simulink model "tb_gnc_mission"  (R2026b)
settings: Solver=ode3  StopTime=10  FixedStep=1e-3  EnableMultiTasking=on
values from neighbouring files (symbols this model uses):
  cmd = y.get('gnc_cmd').Values    [gnc_mission_run.m]    (also in gnc_tb_run.m; t_gnc_mission.m = [1 2; 14 4; 26 5; 27 2; 32 7; 35 7])
  map = P.ic.Bus_TebMapInfo    [t_gnc_mission.m]    (also in t_t07_gnc_sil.m = struct())
  P = F.P    [gnc_fsm_driver.m]    (also in t_gnc_mission.m = r.P; t_t07_gnc_sil.m = shaddad_params('World', 3, 'Assign', false))
  Ts = pr.Ts    [t_gnc_mission.m]
undefined symbols (not defined in the file or in its folder): aligned, angles_B, bms_critical, charging, cmd_seq, DiscIntNeverNeededParam, drive_ready, estop_active, eul, gnssFixType, headingValid, heartbeat, implement_ready, implement_type, magnitude, navValid, pos_W, posStd, power_ready, protectiveStop, protFieldLen, quality, ranges_B, rc_link_ok, rc_mode_sw, scanValid, section_mask, SOC, t_scan, target_density, v_applied, v_track_meas, valid, vel_B, yawRate
libraries: simulink x15, robotmobilelib x1
settings Model: Creator=aomar  LastModifiedBy=aomar
settings ConfigSet: Description=Shaddad fixed-step 1 ms ode3, multitasking, explicit rate transitions (arch 7, D58).
settings OptimizationCC: SimCompilerOptimization=on
settings DebuggingCC: AlgebraicLoopMsg=error  ArtificialAlgebraicLoopMsg=error  SingleTaskRateTransMsg=error  StrictBusMsg=ErrorOnBusTreatedAsVector
settings SimscapeCC: SimscapeNominalValues="[{\"value\":\"1\",\"unit\":\"A\"},{\"value\":\"1\",\"unit\":\"bar\"},{\"value\":\"1\",\"unit\":\"cm^2\"},{\"value\":\"1\",\"unit\":\"cm^3/s\"},{\"value\":\"1\",\"unit\":\"kJ/kg\"},{\"value\":\"1\",\"unit\":\"kW\"},{\"value\":\"1\",\"unit\":\"l\"},{\"value\":\"1\",\"unit\":\"N\"},{\"value\":\"1\",\"unit\":\"N*m\"},{\"value\":\"1\",\"unit\":\"V\"},{\"value\":\"0.001\",\"unit\":\"Wb\"}]"  SimscapeNormalizeSystem=off  SimscapeUseEnergyAccounting=off

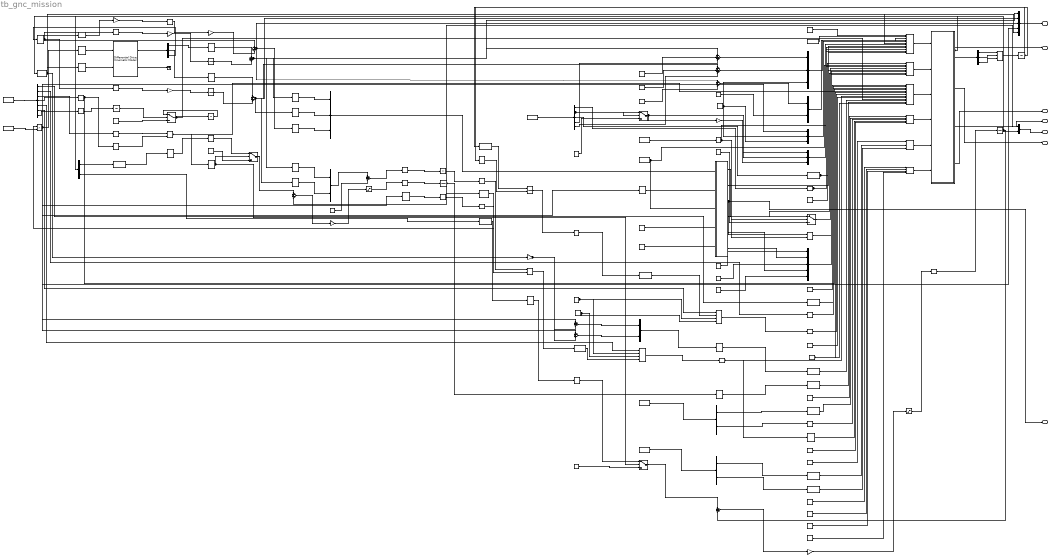
== system tb_gnc_mission ==
  BmsIC : Constant  Value=P.ic.Bus_BmsStatus  OutDataTypeStr=Bus: Bus_BmsStatus  SampleTime=Ts.hk
  BmsStatus : BusAssignment  AssignedSignals=SOC,bms_critical,charging,valid
  CmdIC : Constant  Value=P.ic.Bus_MissionCmd  OutDataTypeStr=Bus: Bus_MissionCmd  SampleTime=Ts.mcmd
  CmdSel : BusSelector  OutputSignals=v_cmd,omega_cmd
  GNC : ModelReference  ModelNameDialog=Shaddad_GNC  SimulationMode=Normal  ModelReferenceVersion=1.1
  HarnessLidar : MATLAB Function  TreatAsAtomicUnit=on  mask{prm=struct('res',P.world.occ.res,'origin',P.world.occ.origin,'rmin',P.sensors.lidar.rMin,'rmax',P.gnc.tb.lidar_rmax,'nBeams',P.gnc.obs.n_beams,'on',P.gnc.tb.lidar_on,'protXF',P.sensors.per.protXF,'protXR',P.sensors.per.protXR,'protL0',P.sensors.per.protL0,'protKv',P.sensors.per.protKv,'protW',P.sensors.per.protW,'protStatic',P.gnc.tb.prot_static,'mapN',P.gnc.map.local_N,'mapRes',P.gnc.map.local_res)}
  ImplSel : BusSelector  OutputSignals=mower_enable,tiller_enable,spray_enable
  Kinematics : robotmobilelib/Differential Drive Kinematic Model  VehicleInputs=Vehicle Speed & Heading Angular Velocity  WheelRadius=P.structure.r_sprocket  WheelSpeedRange=[-inf inf]  TrackWidth=P.structure.geom.B  InitialState=P.gnc.tb.x0(:)  SimulateUsing=Code generation
  Kv : Gain  Gain=P.electronics.shaper.K_v
  Kw : Gain  Gain=P.electronics.shaper.K_w_auto
  Map : BusCreator  Inputs=5  OutDataTypeStr=Bus: Bus_TebMapInfo  NonVirtualBus=on
  McuIC : Constant  Value=P.ic.Bus_McuStatus  OutDataTypeStr=Bus: Bus_McuStatus  SampleTime=Ts.gnc
  McuStatus : BusAssignment  AssignedSignals=rc_mode_sw,rc_link_ok,estop_active,drive_ready,power_ready,implement_ready,charging,implement_type,heartbeat,v_track_meas,v_applied,valid
  MissionCmd : BusAssignment  AssignedSignals=cmd,cmd_seq
  NavIC : Constant  Value=P.ic.Bus_NavState  OutDataTypeStr=Bus: Bus_NavState  SampleTime=Ts.ctrl
  NavState : BusAssignment  AssignedSignals=t,pos_W,eul,vel_B,yawRate,posStd,quality,navValid,headingValid,aligned,gnssFixType
  PerIC : Constant  Value=P.ic.Bus_Perception  OutDataTypeStr=Bus: Bus_Perception  SampleTime=Ts.lidar
  Perception : BusAssignment  AssignedSignals=t_scan,scanValid,ranges_B,angles_B,protectiveStop,protFieldLen,map
  RT_chg : RateTransition  OutPortSampleTime=Ts.hk
  RT_drive : RateTransition  OutPortSampleTime=Ts.ctrl
  RT_ppsi : RateTransition  OutPortSampleTime=Ts.lidar
  RT_pv : RateTransition  OutPortSampleTime=Ts.lidar
  RT_px : RateTransition  OutPortSampleTime=Ts.lidar
  RT_py : RateTransition  OutPortSampleTime=Ts.lidar
  RT_rc : RateTransition  OutPortSampleTime=0
  RT_v : RateTransition  OutPortSampleTime=Ts.ctrl
  RT_vLR : RateTransition  OutPortSampleTime=Ts.gnc
  RT_vapp : RateTransition  OutPortSampleTime=Ts.gnc
  RT_vc : RateTransition  OutPortSampleTime=0
  RT_vd : RateTransition  OutPortSampleTime=Ts.gnc
  RT_w : RateTransition  OutPortSampleTime=Ts.ctrl
  RT_xd : RateTransition  OutPortSampleTime=Ts.gnc
  RT_yd : RateTransition  OutPortSampleTime=Ts.gnc
  Spray : BusAssignment  AssignedSignals=section_mask,target_density,valid
  SprayIC : Constant  Value=P.ic.Bus_SprayDemand  OutDataTypeStr=Bus: Bus_SprayDemand  SampleTime=Ts.spray
  T_stateDot : Terminator
  ZOH_psi : RateTransition  OutPortSampleTime=Ts.ctrl
  ZOH_x : RateTransition  OutPortSampleTime=Ts.ctrl
  ZOH_y : RateTransition  OutPortSampleTime=Ts.ctrl
  a_sat : Saturate  UpperLimit=P.electronics.shaper.a_acc_auto  LowerLimit=-P.electronics.shaper.a_dec_auto
  al_sat : Saturate  UpperLimit=P.electronics.shaper.alpha_auto  LowerLimit=-P.electronics.shaper.alpha_auto
  at_dock : Logic  AllPortsSameDT=off  OutDataTypeStr=boolean
  at_dock_d : DataTypeConversion  OutDataTypeStr=double  RndMeth=Nearest
  bms_crit : simulink/Logic and Bit Operations/Compare To Constant  relop=>  const=0.5  OutDataTypeStr=boolean
  bms_d : Demux  Outputs=2
  bms_true : Constant  Value=true  OutDataTypeStr=boolean  SampleTime=Ts.hk
  charging : simulink/Logic and Bit Operations/Compare To Constant  relop=>  const=0.5  OutDataTypeStr=boolean
  chg_m : MultiPortSwitch  DataPortOrder=Zero-based contiguous  DiagnosticForDefault=None  zeroidx=on  SaturateOnIntegerOverflow=off  InputSameDT=off
  clock : DigitalClock  SampleTime=Ts.ctrl
  clock_l : DigitalClock  SampleTime=Ts.lidar
  cmd_d : Demux  Outputs=2
  cmd_u8 : DataTypeConversion  OutDataTypeStr=uint8  RndMeth=Nearest
  cmd_v : DataTypeConversion  OutDataTypeStr=double  RndMeth=Nearest
  cmd_w : DataTypeConversion  OutDataTypeStr=double  RndMeth=Nearest
  cos_psi : Trigonometry  Operator=cos
  ddock : Sum  Inputs=+-
  ddock2 : Math  Operator=magnitude^2
  ddock_s : Sum  Inputs=+
  dead_v : Delay  DelayLength=P.gnc.tb.n_dead  InitialCondition=0  SampleTime=Ts.ctrl
  dead_w : Delay  DelayLength=P.gnc.tb.n_dead  InitialCondition=0  SampleTime=Ts.ctrl
  dock_xy : Constant  Value=P.gnc.mission.dock(1:2)  OutDataTypeStr=double  SampleTime=Ts.gnc
  drift_x : Gain  Gain=-P.gnc.tb.drift
  drift_y : Gain  Gain=P.gnc.tb.drift
  drive_ok : Logic  AllPortsSameDT=off  OutDataTypeStr=boolean
  drv_rdy : simulink/Logic and Bit Operations/Compare To Constant  relop=>  const=0.5  OutDataTypeStr=boolean
  dx : DiscreteIntegrator  SampleTime=Ts.ctrl  ICPrevOutput=DiscIntNeverNeededParam  ICPrevScaledInput=DiscIntNeverNeededParam
  dy : DiscreteIntegrator  SampleTime=Ts.ctrl  ICPrevOutput=DiscIntNeverNeededParam  ICPrevScaledInput=DiscIntNeverNeededParam
  dyn : Constant  Value=P.gnc.tb.dyn  OutDataTypeStr=double
  estop : simulink/Logic and Bit Operations/Compare To Constant  relop=>  const=0.5  OutDataTypeStr=boolean
  eul : Mux  Inputs=[1 2]
  ev : Sum  Inputs=+-
  ew : Sum  Inputs=+-
  f0 : Constant  Value=0  OutDataTypeStr=double  SampleTime=Ts.gnc
  f1 : Constant  OutDataTypeStr=double  SampleTime=Ts.gnc
  freeze : simulink/Logic and Bit Operations/Compare To Constant  relop=>  const=0.5  OutDataTypeStr=boolean
  freeze_z : UnitDelay  InitialCondition=false  SampleTime=Ts.gnc
  gate_v : Switch  Criteria=u2 ~= 0  SaturateOnIntegerOverflow=off  InputSameDT=off
  gate_w : Switch  Criteria=u2 ~= 0  SaturateOnIntegerOverflow=off  InputSameDT=off
  hb : Switch  Criteria=u2 ~= 0  SaturateOnIntegerOverflow=off  InputSameDT=off
  hb_cnt : simulink/Sources/Counter Free-Running  NumBits=8  tsamp=Ts.gnc
  hb_z : UnitDelay  InitialCondition=uint8(0)  SampleTime=Ts.gnc
  impl_en : Logic  Operator=OR  Inputs=3  AllPortsSameDT=off  OutDataTypeStr=boolean
  impl_en_d : DataTypeConversion  OutDataTypeStr=double  RndMeth=Nearest
  impl_en_z : UnitDelay  InitialCondition=false  SampleTime=Ts.gnc
  impl_off : Logic  Operator=NOT  Inputs=1  AllPortsSameDT=off  OutDataTypeStr=boolean
  impl_rdy : simulink/Logic and Bit Operations/Compare To Constant  relop=>  const=0.5  OutDataTypeStr=boolean
  impl_rdy_m : MultiPortSwitch  DataPortOrder=Zero-based contiguous  DiagnosticForDefault=None  zeroidx=on  SaturateOnIntegerOverflow=off  InputSameDT=off
  impl_type : Constant  Value=P.gnc.mission.implement_type  OutDataTypeStr=uint8  SampleTime=Ts.gnc
  jerk_v : RateLimiter  RisingSlewLimit=P.electronics.shaper.j_max  FallingSlewLimit=-P.electronics.shaper.j_max  SampleTimeMode=inherited
  jerk_w : RateLimiter  RisingSlewLimit=P.electronics.shaper.jw_auto  FallingSlewLimit=-P.electronics.shaper.jw_auto  SampleTimeMode=inherited
  lag_r : simulink/Discrete/Transfer Fcn First Order  PoleZ=exp(-Ts.ctrl/P.gnc.tb.tau_r)  ICPrevOutput=0.0  DoSatur=off
  lag_v : simulink/Discrete/Transfer Fcn First Order  PoleZ=exp(-Ts.ctrl/P.gnc.tb.tau_v)  ICPrevOutput=0.0  DoSatur=off
  map_org : Constant  Value=-[1 1]*P.gnc.map.local_N/(2*P.gnc.map.local_res)  VectorParams1D=off  OutDataTypeStr=double  SampleTime=Ts.lidar
  map_res : Constant  Value=P.gnc.map.local_res  OutDataTypeStr=double  SampleTime=Ts.lidar
  map_size : Constant  Value=[1 1]*P.gnc.map.local_N  VectorParams1D=off  OutDataTypeStr=double  SampleTime=Ts.lidar
  mcu_d : Demux  Outputs=7
  mcu_true : Constant  Value=true  OutDataTypeStr=boolean  SampleTime=Ts.gnc
  n_psi : RandomNumber  Variance=P.gnc.tb.sig_yaw^2  Seed=P.gnc.tb.seed_psi  SampleTime=Ts.ctrl
  n_x : RandomNumber  Variance=P.gnc.tb.sig_pos^2  Seed=P.gnc.tb.seed_x  SampleTime=Ts.ctrl
  n_y : RandomNumber  Variance=P.gnc.tb.sig_pos^2  Seed=P.gnc.tb.seed_y  SampleTime=Ts.ctrl
  nan_r : Constant  Value=NaN(P.gnc.obs.n_beams, 1)  OutDataTypeStr=single  SampleTime=Ts.lidar
  nav_d : Demux  Outputs=5
  near_dock : simulink/Logic and Bit Operations/Compare To Constant  relop=<  const=P.gnc.tb.dock_tol^2  OutDataTypeStr=boolean
  no_estop : Logic  Operator=NOT  Inputs=1  AllPortsSameDT=off  OutDataTypeStr=boolean
  occ : Constant  Value=P.world.occ.grid  OutDataTypeStr=boolean
  posStd : Mux  Inputs=3
  pos_W : Mux  Inputs=3
  pose_l : Mux  Inputs=3
  prot_v : Logic  AllPortsSameDT=off  OutDataTypeStr=boolean
  psi_2pi : Gain  Gain=2*pi
  psi_b : Bias  Bias=pi  SaturateOnIntegerOverflow=off
  psi_f : Rounding
  psi_meas : Sum
  psi_n : Gain  Gain=1/(2*pi)
  psi_w : Sum  Inputs=+-
  quality : DataTypeConversion  OutDataTypeStr=uint8  RndMeth=Nearest
  ranges_v : Switch  Criteria=u2 ~= 0  SaturateOnIntegerOverflow=off  InputSameDT=off
  rc_link : simulink/Logic and Bit Operations/Compare To Constant  relop=>  const=0.5  OutDataTypeStr=boolean
  rc_sw : DataTypeConversion  OutDataTypeStr=uint8  RndMeth=Nearest
  scan_ok : simulink/Logic and Bit Operations/Compare To Constant  relop=>  const=0.5  OutDataTypeStr=boolean
  scn_bms : FromWorkspace  VariableName=P.gnc.tb.scn_bms  SampleTime=Ts.hk  OutputAfterFinalValue=Holding final value
  scn_cmd : FromWorkspace  VariableName=P.gnc.tb.scn_cmd  SampleTime=Ts.mcmd  Interpolate=off  OutputAfterFinalValue=Holding final value
  scn_mcu : FromWorkspace  VariableName=P.gnc.tb.scn_mcu  SampleTime=Ts.gnc  Interpolate=off  OutputAfterFinalValue=Holding final value
  scn_nav : FromWorkspace  VariableName=P.gnc.tb.scn_nav  SampleTime=Ts.ctrl  Interpolate=off  OutputAfterFinalValue=Holding final value
  scn_plant : FromWorkspace  VariableName=P.gnc.tb.scn_plant  SampleTime=Ts.ctrl  Interpolate=off  OutputAfterFinalValue=Holding final value
  scn_scan : FromWorkspace  VariableName=P.gnc.tb.scn_scan  SampleTime=Ts.lidar  Interpolate=off  OutputAfterFinalValue=Holding final value
  seq_u8 : DataTypeConversion  OutDataTypeStr=uint8  RndMeth=Nearest
  shaped_mux : Mux  Inputs=2
  sig : Switch  Criteria=u2 > Threshold  SaturateOnIntegerOverflow=off  InputSameDT=off
  sig_nom : Constant  Value=P.gnc.tb.sig_pos  OutDataTypeStr=double  SampleTime=Ts.ctrl
  sig_z : Gain  Gain=2
  sin_psi : Trigonometry
  soc_s : DataTypeConversion  OutDataTypeStr=single  RndMeth=Nearest
  spin_t : DiscreteIntegrator  ExternalReset=level  SampleTime=Ts.gnc  ICPrevOutput=DiscIntNeverNeededParam  ICPrevScaledInput=DiscIntNeverNeededParam
  spr_dens : Constant  Value=single(P.gnc.tb.spray_density)  OutDataTypeStr=single  SampleTime=Ts.spray
  spr_mask : Constant  Value=uint16(P.gnc.tb.spray_mask)  OutDataTypeStr=uint16  SampleTime=Ts.spray
  spr_valid : Constant  Value=true  OutDataTypeStr=boolean  SampleTime=Ts.spray
  spun : simulink/Logic and Bit Operations/Compare To Constant  relop=>=  const=P.gnc.tb.t_spin  OutDataTypeStr=boolean
  spun_d : DataTypeConversion  OutDataTypeStr=double  RndMeth=Nearest
  state : Demux  Outputs=3
  stopped : simulink/Logic and Bit Operations/Compare To Constant  relop=<  const=0.05  OutDataTypeStr=boolean
  tilt : Constant  Value=P.gnc.tb.tilt(:)  OutDataTypeStr=double  SampleTime=Ts.ctrl
  truth_mux : Mux  Inputs=5
  vL : Sum  Inputs=+-
  vLR : Mux  Inputs=2
  vLR_s : DataTypeConversion  OutDataTypeStr=single  RndMeth=Nearest
  vR : Sum
  v_abs : Abs  SaturateOnIntegerOverflow=off
  v_ref : DiscreteIntegrator  SampleTime=Ts.ctrl  ICPrevOutput=DiscIntNeverNeededParam  ICPrevScaledInput=DiscIntNeverNeededParam
  v_true : Product  Inputs=**
  valid : simulink/Logic and Bit Operations/Compare To Constant  relop=>  const=0.5  OutDataTypeStr=boolean
  vapp_s : DataTypeConversion  OutDataTypeStr=single  RndMeth=Nearest
  vel_B : Mux  Inputs=3
  w_ref : DiscreteIntegrator  SampleTime=Ts.ctrl  ICPrevOutput=DiscIntNeverNeededParam  ICPrevScaledInput=DiscIntNeverNeededParam
  w_track : Gain  Gain=P.electronics.mix.chi*P.electronics.mix.B/2
  x_meas : Sum  Inputs=+++
  x_true : Sum
  xy_t : Mux  Inputs=2
  y_meas : Sum  Inputs=+++
  y_true : Sum
  z_v : Constant  Value=0  OutDataTypeStr=double  SampleTime=Ts.ctrl
  z_w : Constant  Value=0  OutDataTypeStr=double  SampleTime=Ts.ctrl
  zero : Constant  Value=0  OutDataTypeStr=double  SampleTime=Ts.ctrl
  truth : Outport
  gnc_cmd : Outport  Port=2
  gnc_debug : Outport  Port=3
  gnc_status : Outport  Port=4
  shaped : Outport  Port=5
  nav_cmd : Outport  Port=6
  prot : Outport  Port=7
  wires:
  scn_mcu/1 -> mcu_d/1  "scn_mcu"
  scn_plant/1 -> v_true/2  "scn_plant"
  mcu_d/1 -> rc_sw/1  "scn_rc_sw"
  mcu_d/2 -> rc_link/1  "scn_rc_link"
  mcu_d/3 -> drv_rdy/1  "scn_drive_ready"
  mcu_d/4 -> estop/1  "scn_estop"
  mcu_d/5 -> chg_m/1  "scn_charging"
  mcu_d/6 -> impl_rdy_m/1  "scn_impl_ready"
  mcu_d/7 -> freeze/1  "scn_freeze"
  v_true/1 -> vR/1, vL/1, truth_mux/4, RT_vc/1, RT_vd/1, RT_pv/1, vel_B/1  "v_true"
  ZOH_psi/1 -> cos_psi/1, sin_psi/1, psi_w/1, psi_b/1  "ZOH_psi"
  lag_r/1 -> w_track/1, truth_mux/5, NavState/6, RT_rc/1  "r_true"
  CmdSel/1 -> cmd_v/1  "<v_cmd>"
  CmdSel/2 -> cmd_w/1  "<omega_cmd>"
  estop/1 -> no_estop/1, McuStatus/4  "estop"
  freeze/1 -> freeze_z/1  "freeze"
  psi_b/1 -> psi_n/1  "psi_b"
  RT_vc/1 -> Kinematics/1  "RT_vc"
  RT_rc/1 -> Kinematics/2  "RT_rc"
  psi_n/1 -> psi_f/1  "psi_n"
  sin_psi/1 -> drift_x/1  "sin_psi"
  cos_psi/1 -> drift_y/1  "cos_psi"
  hb_cnt/1 -> hb/3  "hb_cnt"
  drv_rdy/1 -> drive_ok/1  "drv_rdy"
  no_estop/1 -> drive_ok/2  "no_estop"
  freeze_z/1 -> hb/2  "freeze_z"
  cmd_v/1 -> RT_v/1  "cmd_v"
  Kinematics/1 -> state/1  "state"
  Kinematics/2 -> T_stateDot/1  "state_dot"
  state/1 -> ZOH_x/1  "state_1"
  state/2 -> ZOH_y/1  "state_2"
  state/3 -> ZOH_psi/1  "state_3"
  psi_f/1 -> psi_2pi/1  "psi_f"
  drift_x/1 -> dx/1  "drift_x"
  drift_y/1 -> dy/1  "drift_y"
  drive_ok/1 -> McuStatus/5, RT_drive/1  "drive_ok"
  RT_v/1 -> dead_v/1  "RT_v"
  hb/1 -> McuStatus/10, hb_z/1  "hb"
  psi_2pi/1 -> psi_w/2  "psi_2pi"
  z_v/1 -> gate_v/3  "z_v"
  dx/1 -> x_true/2  "dx"
  dy/1 -> y_true/2  "dy"
  hb_z/1 -> hb/1  "hb_z"
  dead_v/1 -> gate_v/1  "dead_v"
  ZOH_x/1 -> x_true/1  "ZOH_x"
  ZOH_y/1 -> y_true/1  "ZOH_y"
  RT_drive/1 -> gate_w/2, gate_v/2  "RT_drive"
  x_true/1 -> RT_xd/1, truth_mux/1, RT_px/1, x_meas/1  "x"
  y_true/1 -> RT_yd/1, truth_mux/2, y_meas/1, RT_py/1  "y"
  psi_w/1 -> RT_ppsi/1, psi_meas/1, truth_mux/3  "psi_w"
  gate_v/1 -> ev/1  "gate_v"
  ev/1 -> Kv/1  "ev"
  RT_px/1 -> pose_l/1  "RT_px"
  RT_py/1 -> pose_l/2  "RT_py"
  RT_ppsi/1 -> pose_l/3  "RT_ppsi"
  RT_xd/1 -> xy_t/1  "RT_xd"
  RT_yd/1 -> xy_t/2  "RT_yd"
  pose_l/1 -> HarnessLidar/1(pose)  "pose_l"
  xy_t/1 -> ddock/1  "xy_t"
  dock_xy/1 -> ddock/2  "dock_xy"
  Kv/1 -> a_sat/1  "Kv"
  ddock/1 -> ddock2/1  "ddock"
  a_sat/1 -> jerk_v/1  "a_sat"
  ddock2/1 -> ddock_s/1  "ddock2"
  jerk_v/1 -> v_ref/1  "jerk_v"
  RT_vd/1 -> v_abs/1  "RT_vd"
  ddock_s/1 -> near_dock/1  "ddock_s"
  v_abs/1 -> stopped/1  "v_abs"
  v_ref/1 -> RT_vapp/1, shaped_mux/1, ev/2, lag_v/1  "v_ref"
  impl_off/1 -> spin_t/2  "impl_off"
  near_dock/1 -> at_dock/1  "near_dock"
  stopped/1 -> at_dock/2  "stopped"
  lag_v/1 -> v_true/1  "lag_v"
  impl_en_d/1 -> spin_t/1  "impl_en_d"
  cmd_w/1 -> RT_w/1  "cmd_w"
  w_track/1 -> vR/2, vL/2  "w_track"
  at_dock/1 -> at_dock_d/1  "at_dock"
  spin_t/1 -> spun/1  "spin_t"
  RT_w/1 -> dead_w/1  "RT_w"
  scn_nav/1 -> nav_d/1  "scn_nav"
  nav_d/1 -> valid/1  "scn_valid"
  nav_d/2 -> sig/2, sig/1  "scn_sigma"
  nav_d/3 -> quality/1  "scn_quality"
  nav_d/4 -> x_meas/3  "scn_dx"
  nav_d/5 -> y_meas/3  "scn_dy"
  vL/1 -> vLR/1  "vL"
  vR/1 -> vLR/2  "vR"
  sig_nom/1 -> sig/3  "sig_nom"
  spun/1 -> spun_d/1  "spun"
  f0/1 -> chg_m/2, impl_rdy_m/3  "f0"
  z_w/1 -> gate_w/3  "z_w"
  dead_w/1 -> gate_w/1  "dead_w"
  f1/1 -> chg_m/3, impl_rdy_m/4  "f1"
  at_dock_d/1 -> chg_m/4  "at_dock_d"
  vLR/1 -> RT_vLR/1  "vLR"
  n_x/1 -> x_meas/2  "n_x"
  n_y/1 -> y_meas/2  "n_y"
  n_psi/1 -> psi_meas/2  "n_psi"
  occ/1 -> HarnessLidar/4(occ)  "occ"
  dyn/1 -> HarnessLidar/5(dyn)  "dyn"
  chg_m/1 -> charging/1  "chg"
  RT_pv/1 -> HarnessLidar/2(v)  "RT_pv"
  sig/1 -> posStd/2, posStd/1, sig_z/1  "sig"
  gate_w/1 -> ew/1  "gate_w"
  scn_scan/1 -> scan_ok/1  "scn_scan"
  clock_l/1 -> Perception/2, HarnessLidar/3(t)  "clock_l"
  scn_bms/1 -> bms_d/1  "scn_bms"
  scn_cmd/1 -> cmd_d/1  "scn_cmd"
  spun_d/1 -> impl_rdy_m/2  "spun_d"
  bms_d/1 -> soc_s/1  "scn_soc"
  bms_d/2 -> bms_crit/1  "scn_bms_crit"
  cmd_d/1 -> cmd_u8/1  "scn_cmd"
  cmd_d/2 -> seq_u8/1  "scn_seq"
  x_meas/1 -> pos_W/1  "x_meas"
  y_meas/1 -> pos_W/2  "y_meas"
  psi_meas/1 -> eul/1  "psi_meas"
  ew/1 -> Kw/1  "ew"
  tilt/1 -> eul/2  "tilt"
  sig_z/1 -> posStd/3  "sig_z"
  scan_ok/1 -> prot_v/2, ranges_v/2, Perception/3  "scan_ok"
  nan_r/1 -> ranges_v/3  "nan_r"
  map_res/1 -> Map/1  "Resolution"
  map_size/1 -> Map/3  "GridSize"
  map_org/1 -> Map/5  "GridOriginInLocal"
  impl_rdy_m/1 -> impl_rdy/1  "impl_rdy"
  zero/1 -> vel_B/3, vel_B/2, pos_W/3  "zero"
  RT_vLR/1 -> vLR_s/1  "RT_vLR"
  RT_vapp/1 -> vapp_s/1  "RT_vapp"
  charging/1 -> McuStatus/8, RT_chg/1  "charging"
  HarnessLidar/1(ranges) -> ranges_v/1  "ranges"
  HarnessLidar/2(angles) -> Perception/5  "angles"
  HarnessLidar/3(prot) -> prot/1, prot_v/1  "prot"
  HarnessLidar/4(protLen) -> Perception/7  "protLen"
  HarnessLidar/5(occL) -> Map/4  "OccupancyMatrix"
  HarnessLidar/6(gl) -> Map/2  "GridLocationInWorld"
  pos_W/1 -> NavState/3  "pos_W"
  eul/1 -> NavState/4  "eul"
  vel_B/1 -> NavState/5  "vel_B"
  posStd/1 -> NavState/7  "posStd"
  Map/1 -> Perception/8  "Map"
  NavIC/1 -> NavState/1  "NavIC"
  valid/1 -> NavState/9, NavState/10, NavState/11  "valid"
  PerIC/1 -> Perception/1  "PerIC"
  prot_v/1 -> Perception/6  "prot_v"
  McuIC/1 -> McuStatus/1  "McuIC"
  rc_link/1 -> McuStatus/3  "rc_link"
  impl_rdy/1 -> McuStatus/7  "impl_rdy"
  impl_type/1 -> McuStatus/9  "impl_type"
  BmsIC/1 -> BmsStatus/1  "BmsIC"
  bms_crit/1 -> BmsStatus/3  "bms_crit"
  bms_true/1 -> BmsStatus/5  "bms_true"
  CmdIC/1 -> MissionCmd/1  "CmdIC"
  SprayIC/1 -> Spray/1  "SprayIC"
  spr_mask/1 -> Spray/2  "spr_mask"
  spr_dens/1 -> Spray/3  "spr_dens"
  spr_valid/1 -> Spray/4  "spr_valid"
  Kw/1 -> al_sat/1  "Kw"
  mcu_true/1 -> McuStatus/6, McuStatus/13  "mcu_true"
  RT_chg/1 -> BmsStatus/4  "RT_chg"
  ranges_v/1 -> Perception/4  "ranges_v"
  clock/1 -> NavState/2  "clock"
  quality/1 -> NavState/8, NavState/12  "quality"
  rc_sw/1 -> McuStatus/2  "rc_sw"
  vLR_s/1 -> McuStatus/11  "vLR_s"
  vapp_s/1 -> McuStatus/12  "vapp_s"
  soc_s/1 -> BmsStatus/2  "soc_s"
  cmd_u8/1 -> MissionCmd/2  "cmd_u8"
  seq_u8/1 -> MissionCmd/3  "seq_u8"
  al_sat/1 -> jerk_w/1  "al_sat"
  NavState/1 -> GNC/1  "nav_state"
  Perception/1 -> GNC/2  "perception"
  McuStatus/1 -> GNC/3  "mcu_status"
  BmsStatus/1 -> GNC/4  "bms_status"
  MissionCmd/1 -> GNC/5  "mcmd"
  Spray/1 -> GNC/6  "spray"
  jerk_w/1 -> w_ref/1  "jerk_w"
  GNC/1 -> CmdSel/1, ImplSel/1, gnc_cmd/1  "gnc_cmd"
  GNC/2 -> nav_cmd/1  "nav_cmd"
  GNC/3 -> gnc_status/1  "gnc_status"
  GNC/4 -> gnc_debug/1  "gnc_debug"
  ImplSel/1 -> impl_en/1  "<mower_enable>"
  ImplSel/2 -> impl_en/2  "<tiller_enable>"
  ImplSel/3 -> impl_en/3  "<spray_enable>"
  impl_en/1 -> impl_en_z/1  "impl_en"
  w_ref/1 -> ew/2, lag_r/1, shaped_mux/2  "w_ref"
  truth_mux/1 -> truth/1  "truth"
  shaped_mux/1 -> shaped/1  "shaped"
  impl_en_z/1 -> impl_off/1, impl_en_d/1  "impl_en_z"

== matlab function tb_gnc_mission/HarnessLidar ==
  settings: updateMethod=DISCRETE  sampleTime=Ts.lidar  description=Harness LiDAR (gnc spec 4.5, tests only); body subsystems/gnc/gnc_harnessLidar.m.
  data: pose input; ranges output; v input; t input; occ input; dyn input; angles output; prot output; protLen output; occL output; gl output; prm parameter
function [ranges, angles, prot, protLen, occL, gl] = fcn(pose, v, t, occ, dyn, prm)
%#codegen
[ranges, angles, prot, protLen, occL, gl] = gnc_harnessLidar(pose, v, t, occ, dyn, prm);
